simulink model "first_lab"  (R2025b)
settings: Solver=ode45  StartTime=0.0  StopTime=20.0  RelTol=1e-3
settings Model: Creator=reino  LastModifiedBy=reino

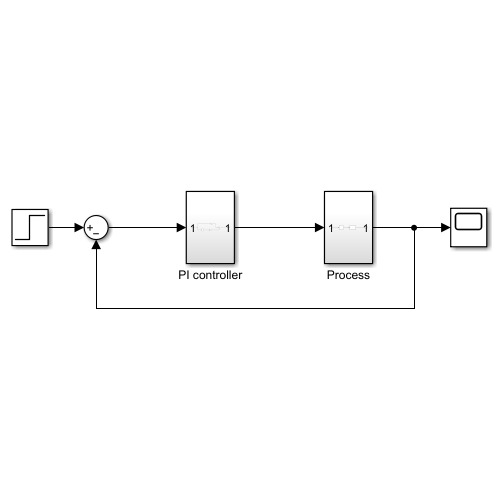
[thumbnail: Simulink's stored preview of the top-level diagram]
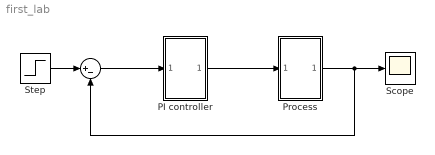
== system first_lab ==
  " " : Sum  Inputs=|+-
  PI controller : Subsystem
  Process : Subsystem
  Scope : Scope
      settings: ActiveDisplayYMinimum=-0.12512874063658377  ActiveDisplayYMaximum=1.1261586657292542
  Step : Step  SampleTime=0
  wires:
  Step/1 -> " "/1
  Process/1(Out2) -> " "/2, Scope/1
  " "/1 -> PI controller/1(In2)
  PI controller/1(Out1) -> Process/1(In1)

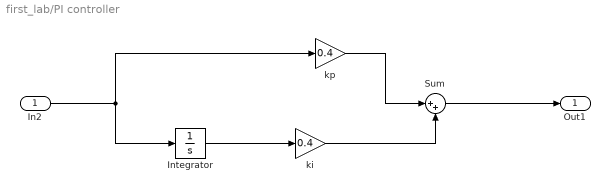
== system first_lab/PI controller ==
  In2 : Inport
  Integrator : Integrator
  Sum : Sum  Inputs=|++
  ki : Gain  Gain=0.4
  kp : Gain  Gain=0.4
  Out1 : Outport
  wires:
  In2/1 -> kp/1, Integrator/1
  ki/1 -> Sum/2
  Sum/1 -> Out1/1
  kp/1 -> Sum/1
  Integrator/1 -> ki/1

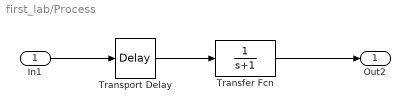
== system first_lab/Process ==
  In1 : Inport
  Transfer Fcn : TransferFcn  Denominator=[1 1]
  Transport Delay : TransportDelay
  Out2 : Outport
  wires:
  Transport Delay/1 -> Transfer Fcn/1
  Transfer Fcn/1 -> Out2/1
  In1/1 -> Transport Delay/1
